simulink model "DCServomotor_Cpy"  (R2024a)
settings: Solver=ode45  StartTime=0.0  StopTime=45  MaxStep=1e-02  RelTol=1e-1
undefined symbols (not defined in the file): degs2rpm, delta_i, gbox, Kd, Ki, Kp, mot, sens, TL, wc, wc2
libraries: simulink x9
settings Model: Creator=liliy  LastModifiedBy=lenovo
settings SolverCC: ZeroCrossAlgorithm=Adaptive
settings DebuggingCC: IgnoredZcDiagnostic=none

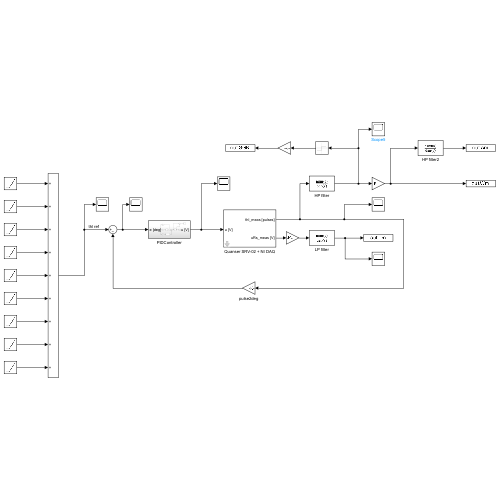
[thumbnail: Simulink's stored preview of the top-level diagram]
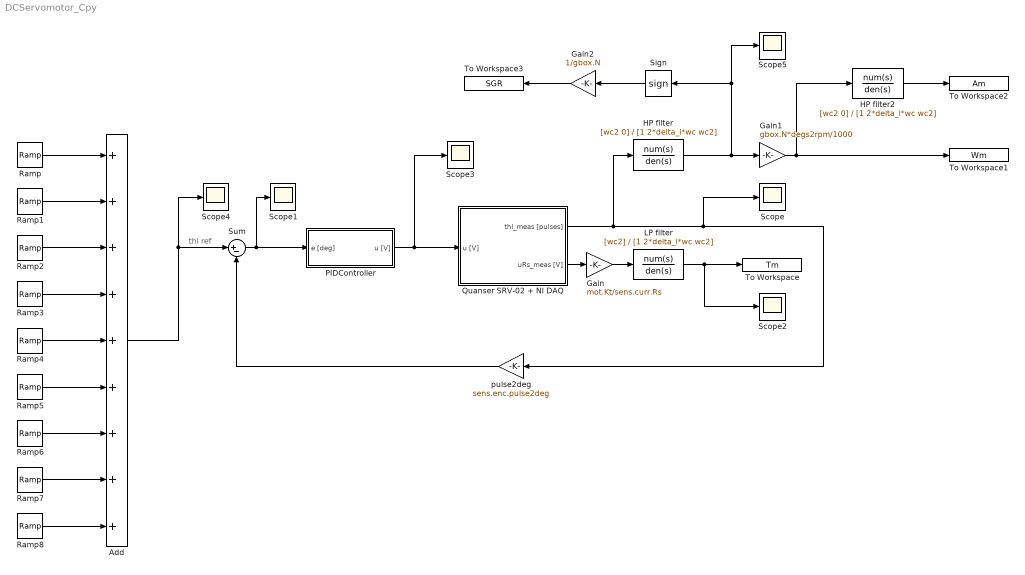
== system DCServomotor_Cpy ==
  note: thl ref
  Add : Sum  Inputs=+++++++++
  Gain : Gain  Gain=mot.Kt/sens.curr.Rs
  Gain1 : Gain  Gain=gbox.N*degs2rpm/1000
  Gain2 : Gain  Gain=1/gbox.N
  HP filter : TransferFcn  Numerator=[wc2 0]  Denominator=[1 2*delta_i*wc wc2]
  HP filter2 : TransferFcn  Numerator=[wc2 0]  Denominator=[1 2*delta_i*wc wc2]
  LP filter : TransferFcn  Numerator=[wc2]  Denominator=[1 2*delta_i*wc wc2]
  PIDController : Subsystem
  Quanser SRV-02 + NI DAQ : Subsystem  mask(Quanser SRV-02 (with inertial load) + NI DAQ){Ts=0.001, fricType=Coulomb + viscous}
      mask prompts: Ts "NI DAQ Sample Time:"; fricType "Friction model"
      mask help: Quanser SRV-02 (with inertial load) + NI DAQ model.
      mask init:
      | %%  Sensors data
      | 
      | %   shunt resistor
      | sens.curr.Rs = 0.5;                         %   resistance [Ohm]   
      | sens.curr.uRs_std = 0.01;                   %   voltage noise standard dev [V]                           
      | sens.curr.uRs_var = sens.curr.uRs_std^2;	%   voltage noise variance [V^2]
      | 
      | %   Hewlett-Packard HEDS-5540#A06 optical encoder
      | sens.enc.ppr = 500*4;                       %   pulses per rotation
      | sens.enc.pulse2deg = 360/sens.enc.ppr;      %   [pulses] -> [deg]
      | sens.enc.pulse2rad = 2*pi/sens.enc.ppr;     %   [pulses] -> [rad]
      | sens.enc.deg2pulse = sens.enc.ppr/360;      %   [deg] -> [pulses]
      | sens.enc.rad2pulse = sens.enc.ppr/2/pi;     %   [rad] -> [pulses]
      | 
      | 
      | %%  Data acquisition board (daq) data
      | 
      | %   NI PCI-6221 DAC data
      | daq.dac.bits = 16;                                  %   resolution (bits)
      | daq.dac.fs   = 10;                                  %   full scale 
      | daq.dac.q    = 2*daq.dac.fs/(2^daq.dac.bits-1);     %	quantization
      | 
      | %   NI PCI-6221 ADC data
      | daq.adc.bits = 16;                                  %   resolution (bits)
      | daq.adc.fs   = 10;                                  %   full scale (as set in SLDRT Analog Input block)
      | daq.adc.q    = 2*daq.adc.fs/(2^daq.adc.bits-1);     %   quantization
      mask Help:
      | Riccardo Antonello (antonello@dei.unipd.it)
      | 
      | April 24, 2020
      | 
      | Dept. of Information Engineering, University of Padova
      mask TypeOptions fricType: Coulomb + viscous | Karnopp
  Ramp : simulink/Sources/Ramp  slope=300  start=0  InitialOutput=0
  Ramp1 : simulink/Sources/Ramp  slope=300  start=5  InitialOutput=0
  Ramp2 : simulink/Sources/Ramp  slope=300  start=10  InitialOutput=0
  Ramp3 : simulink/Sources/Ramp  slope=300  start=15  InitialOutput=0
  Ramp4 : simulink/Sources/Ramp  slope=300  start=20  InitialOutput=0
  Ramp5 : simulink/Sources/Ramp  slope=300  start=25  InitialOutput=0
  Ramp6 : simulink/Sources/Ramp  slope=300  start=30  InitialOutput=0
  Ramp7 : simulink/Sources/Ramp  slope=300  start=35  InitialOutput=0
  Ramp8 : simulink/Sources/Ramp  slope=300  start=40  InitialOutput=0
  Scope{,1..5} (6 alike) : Scope
  Sign : Signum
  Sum : Sum  Inputs=|+-
  To Workspace : ToWorkspace  VariableName=Tm  SaveFormat=Timeseries  SampleTime=0.1
  To Workspace1 : ToWorkspace  VariableName=Wm  SaveFormat=Timeseries  SampleTime=0.1
  To Workspace2 : ToWorkspace  VariableName=Am  SaveFormat=Timeseries  SampleTime=0.1
  To Workspace3 : ToWorkspace  VariableName=SGR  SaveFormat=Timeseries  SampleTime=0.1
  pulse2deg : Gain  Gain=sens.enc.pulse2deg
  wires:
  pulse2deg/1 -> Sum/2
  Sum/1 -> PIDController/1(e [deg]), Scope1/1
  PIDController/1(u [V]) -> Scope3/1, Quanser SRV-02 + NI DAQ/1(u [V])
  Quanser SRV-02 + NI DAQ/1(thl_meas [pulses]) -> HP filter/1, Scope/1, pulse2deg/1
  Quanser SRV-02 + NI DAQ/2(uRs_meas [V]) -> Gain/1
  Gain/1 -> LP filter/1
  Add/1 -> Scope4/1, Sum/1
  Ramp/1 -> Add/1
  Ramp1/1 -> Add/2
  Ramp2/1 -> Add/3
  Ramp3/1 -> Add/4
  Ramp4/1 -> Add/5
  Ramp5/1 -> Add/6
  Ramp6/1 -> Add/7
  Ramp7/1 -> Add/8
  Ramp8/1 -> Add/9
  LP filter/1 -> Scope2/1, To Workspace/1
  HP filter/1 -> Sign/1, Scope5/1, Gain1/1
  Gain1/1 -> HP filter2/1, To Workspace1/1
  HP filter2/1 -> To Workspace2/1
  Sign/1 -> Gain2/1
  Gain2/1 -> To Workspace3/1

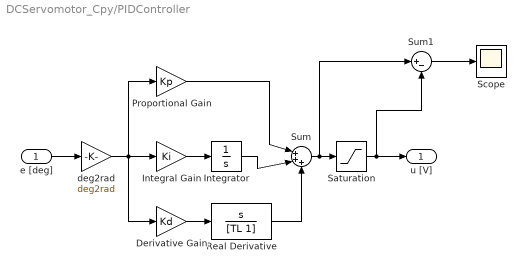
== system DCServomotor_Cpy/PIDController ==
  e [deg] : Inport
  Derivative Gain : Gain  Gain=Kd
  Integral Gain : Gain  Gain=Ki
  Integrator : Integrator
  Proportional Gain : Gain  Gain=Kp
  Real Derivative : TransferFcn  Numerator=[1 0]  Denominator=[TL 1]
  Saturation : Saturate  UpperLimit=12  LowerLimit=-12
  Scope : Scope
  Sum : Sum  Inputs=|+++
  Sum1 : Sum  Inputs=|+-
  deg2rad : Gain  Gain=deg2rad
  u [V] : Outport
  wires:
  Saturation/1 -> Sum1/2, u [V]/1
  Sum/1 -> Sum1/1, Saturation/1
  Real Derivative/1 -> Sum/3
  Sum1/1 -> Scope/1
  Integral Gain/1 -> Integrator/1
  deg2rad/1 -> Derivative Gain/1, Proportional Gain/1, Integral Gain/1
  Integrator/1 -> Sum/2
  e [deg]/1 -> deg2rad/1
  Proportional Gain/1 -> Sum/1
  Derivative Gain/1 -> Real Derivative/1

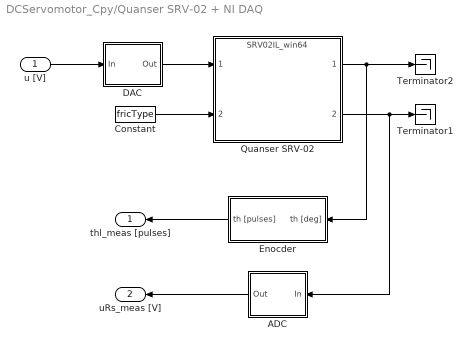
== system DCServomotor_Cpy/Quanser SRV-02 + NI DAQ ==
  u [V] : Inport
  ADC : Subsystem
  Constant : Constant  Value=fricType
  DAC : Subsystem
  Enocder : Subsystem
  Quanser SRV-02 : ModelReference  ModelNameDialog=SRV02IL_win64.slxp  ModelReferenceVersion=1.44  CopyOfModelProtected=on
  Terminator1 : Terminator
  Terminator2 : Terminator
  thl_meas [pulses] : Outport
  uRs_meas [V] : Outport  Port=2
  wires:
  Enocder/1(th [pulses]) -> thl_meas [pulses]/1
  ADC/1(Out) -> uRs_meas [V]/1
  DAC/1(Out) -> Quanser SRV-02/1
  Quanser SRV-02/2 -> ADC/1(In), Terminator1/1
  u [V]/1 -> DAC/1(In)
  Quanser SRV-02/1 -> Enocder/1(th [deg]), Terminator2/1
  Constant/1 -> Quanser SRV-02/2

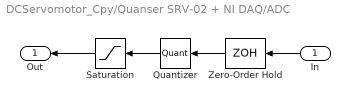
== system DCServomotor_Cpy/Quanser SRV-02 + NI DAQ/ADC ==
  In : Inport
  Quantizer : Quantizer  QuantizationInterval=daq.adc.q
  Saturation : Saturate  UpperLimit=daq.adc.fs  LowerLimit=-daq.adc.fs
  Zero-Order Hold : ZeroOrderHold  SampleTime=Ts
  Out : Outport
  wires:
  Saturation/1 -> Out/1
  In/1 -> Zero-Order Hold/1
  Quantizer/1 -> Saturation/1
  Zero-Order Hold/1 -> Quantizer/1

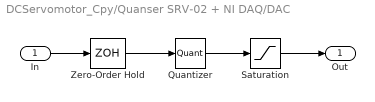
== system DCServomotor_Cpy/Quanser SRV-02 + NI DAQ/DAC ==
  In : Inport
  Quantizer : Quantizer  QuantizationInterval=daq.dac.q
  Saturation : Saturate  UpperLimit=daq.dac.fs  LowerLimit=-daq.dac.fs
  Zero-Order Hold : ZeroOrderHold  SampleTime=Ts
  Out : Outport
  wires:
  Quantizer/1 -> Saturation/1
  In/1 -> Zero-Order Hold/1
  Zero-Order Hold/1 -> Quantizer/1
  Saturation/1 -> Out/1

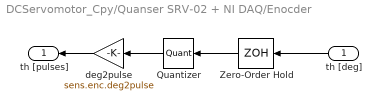
== system DCServomotor_Cpy/Quanser SRV-02 + NI DAQ/Enocder ==
  th [deg] : Inport
  Quantizer : Quantizer  QuantizationInterval=sens.enc.pulse2deg
  Zero-Order Hold : ZeroOrderHold  SampleTime=Ts
  deg2pulse : Gain  Gain=sens.enc.deg2pulse
  th [pulses] : Outport
  wires:
  Quantizer/1 -> deg2pulse/1
  th [deg]/1 -> Zero-Order Hold/1
  Zero-Order Hold/1 -> Quantizer/1
  deg2pulse/1 -> th [pulses]/1
